simulink model "half_car_body"  (R2021b)
settings: Solver=VariableStepAuto  StartTime=0.0  StopTime=10.0  RelTol=1e-3
settings Model: Creator=Emil Chodowiec  LastModifiedBy=Emil Chodowiec

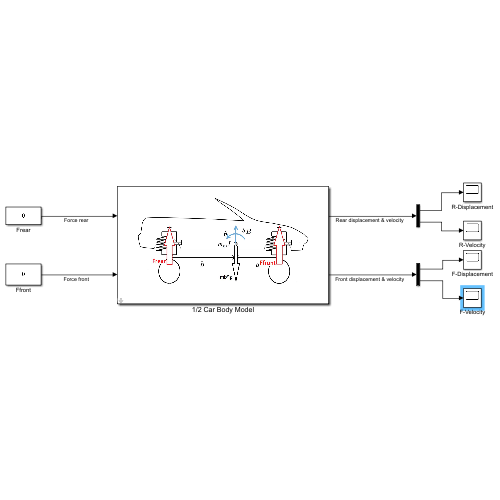
[thumbnail: Simulink's stored preview of the top-level diagram]
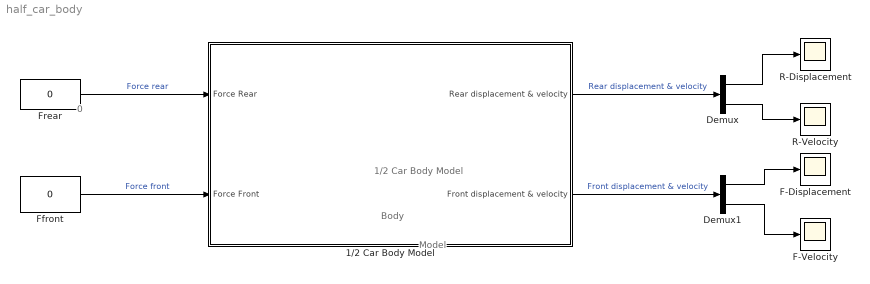
== system half_car_body ==
  note: 0
  note: Body
  note: 1/2 Car Body Model
  note: Model
  1/2 Car Body Model : Subsystem  mask{mb=500, I=600, g=9.81, a=1.25, b=1.4}
      mask prompts: mb "Body mass (mb) [kg]"; I "Inertia (I) [kg/m^2]"; g "Gravitational accelaration (g) [m/s^2]"; a "Length (a) [m]"; b "Length (b) [m]"
      mask DialogControl DescGroupVar Prompt: 1/2 Car Body Model
      mask DialogControl DescTextVar Prompt: Please define vehicle body parameters below.
      mask Display: disp('1/2 car body')
  Demux : Demux  Outputs=2
  Demux1 : Demux  Outputs=2
  F-Displacement : Scope
  F-Velocity : Scope
  Ffront : Constant  Value=0
  Frear : Constant  Value=0
  R-Displacement : Scope
  R-Velocity : Scope
  wires:
  Frear/1 -> 1/2 Car Body Model/1("Force Rear ")  "Force rear"
  Ffront/1 -> 1/2 Car Body Model/2(Force Front)  "Force front"
  1/2 Car Body Model/1(Rear displacement & velocity) -> Demux/1  "Rear displacement & velocity"
  1/2 Car Body Model/2(Front displacement & velocity) -> Demux1/1  "Front displacement & velocity"
  Demux1/1 -> F-Displacement/1
  Demux/1 -> R-Displacement/1
  Demux/2 -> R-Velocity/1
  Demux1/2 -> F-Velocity/1

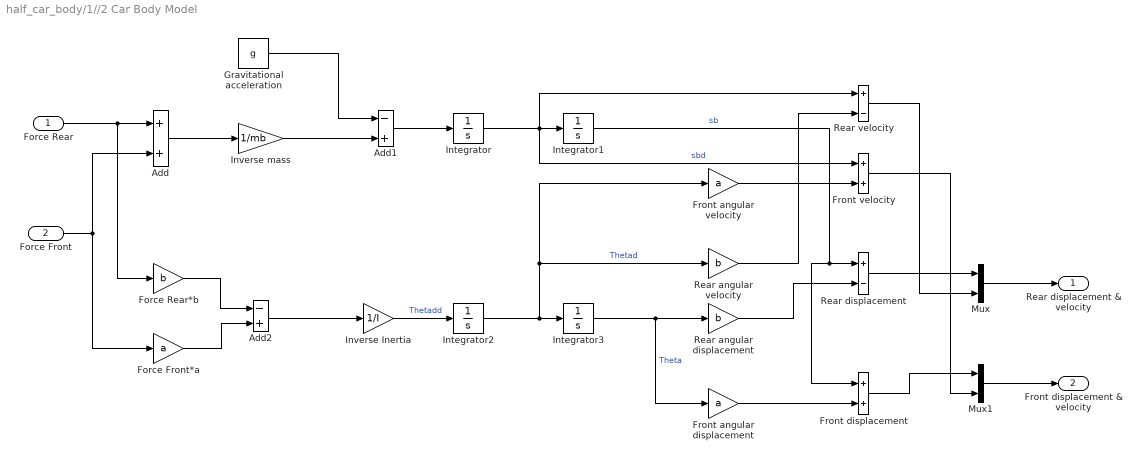
== system half_car_body/1//2 Car Body Model ==
  "Force Rear " : Inport
  Force Front : Inport  Port=2
  Add : Sum
  Add1 : Sum  Inputs=-+
  Add2 : Sum  Inputs=-+
  Force Front*a : Gain  Gain=a
  Force Rear*b : Gain  Gain=b
  Front angular displacement : Gain  Gain=a
  Front angular velocity : Gain  Gain=a
  Front displacement : Sum
  Front velocity : Sum
  Gravitational acceleration : Constant  Value=g
  Integrator{,1..3} (4 alike) : Integrator
  Inverse Inertia : Gain  Gain=1/I
  Inverse mass : Gain  Gain=1/mb
  Mux : Mux  Inputs=2
  Mux1 : Mux  Inputs=2
  Rear angular displacement : Gain  Gain=b
  Rear angular velocity : Gain  Gain=b
  Rear displacement : Sum  Inputs=+-
  Rear velocity : Sum  Inputs=+-
  Rear displacement & velocity : Outport
  Front displacement & velocity : Outport  Port=2
  wires:
  Force Front/1 -> Force Front*a/1, Add/2
  Add/1 -> Inverse mass/1
  Integrator/1 -> Rear velocity/1, Front velocity/1, Integrator1/1  "sbd"
  Gravitational acceleration/1 -> Add1/1
  Inverse mass/1 -> Add1/2
  Add1/1 -> Integrator/1
  Integrator1/1 -> Front displacement/1, Rear displacement/1  "sb"
  Force Front*a/1 -> Add2/2
  Force Rear*b/1 -> Add2/1
  Add2/1 -> Inverse Inertia/1
  Inverse Inertia/1 -> Integrator2/1  "Thetadd"
  Integrator2/1 -> Integrator3/1, Rear angular velocity/1, Front angular velocity/1  "Thetad"
  Integrator3/1 -> Rear angular displacement/1, Front angular displacement/1  "Theta"
  "Force Rear "/1 -> Add/1, Force Rear*b/1
  Rear angular displacement/1 -> Rear displacement/2
  Front angular displacement/1 -> Front displacement/2
  Mux/1 -> Rear displacement & velocity/1
  Mux1/1 -> Front displacement & velocity/1
  Front velocity/1 -> Mux1/2
  Rear displacement/1 -> Mux/1
  Front displacement/1 -> Mux1/1
  Rear velocity/1 -> Mux/2
  Rear angular velocity/1 -> Rear velocity/2
  Front angular velocity/1 -> Front velocity/2
